simulink model "Sandbox"  (R2026b)
settings: Solver=VariableStepAuto  StopTime=20
model workspace (MAT data in the model file):
  MW_MaxNumBodies = 100
  MW_MaxNumCollisions = 5
  MW_MaxNumVertices = 10000
undefined symbols (not defined in the file): K_Lookup, t_s, Tau_Lookup
libraries: simulink x1, embmathops x1
settings Model: Creator=Janelyn Anderson  LastModifiedBy=Janelyn Anderson
settings SimscapeCC: SimscapeLogType=all  SimscapeNominalValues="[{\"value\":\"1\",\"unit\":\"A\"},{\"value\":\"1\",\"unit\":\"bar\"},{\"value\":\"1\",\"unit\":\"cm^2\"},{\"value\":\"1\",\"unit\":\"cm^3/s\"},{\"value\":\"1\",\"unit\":\"kJ/kg\"},{\"value\":\"1\",\"unit\":\"kW\"},{\"value\":\"1\",\"unit\":\"l\"},{\"value\":\"1\",\"unit\":\"N\"},{\"value\":\"1\",\"unit\":\"N*m\"},{\"value\":\"1\",\"unit\":\"V\"},{\"value\":\"0.001\",\"unit\":\"Wb\"}]"  SimscapeUseEnergyAccounting=off

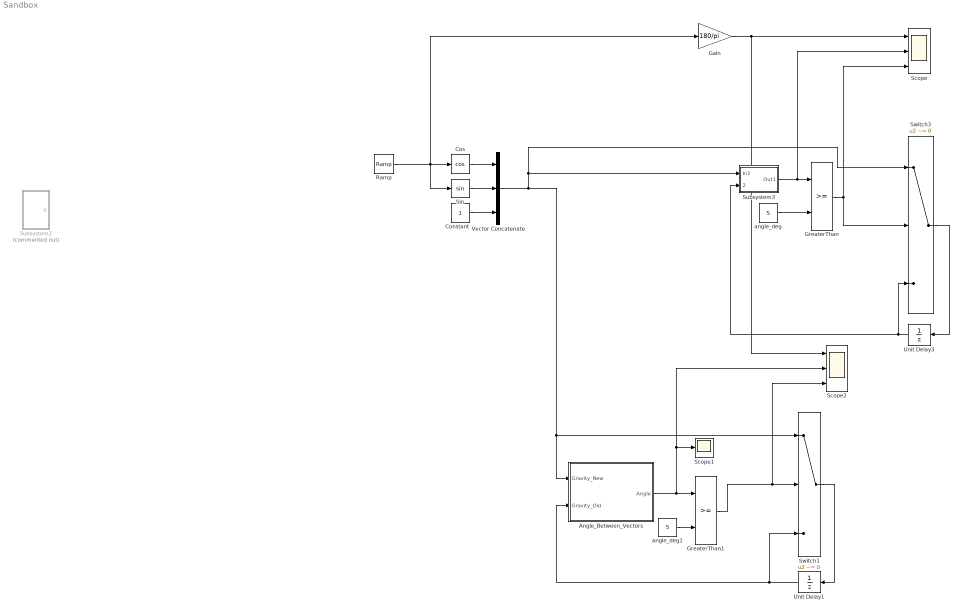
== system Sandbox ==
  Angle_Between_Vectors : Subsystem
  Constant : Constant
  Cos : Trigonometry  Operator=cos
  Gain : Gain  Gain=180/pi
  GreaterThan : RelationalOperator  OutDataTypeStr=boolean  RndMeth=Simplest  InputSameDT=off
  GreaterThan1 : RelationalOperator  OutDataTypeStr=boolean  RndMeth=Simplest  InputSameDT=off
  Ramp : simulink/Sources/Ramp  slope=(10/360)*(2*pi)/20  start=0  InitialOutput=0
  Scope : Scope  NumInputPorts=3
      settings: ActiveDisplayYMinimum=-1.2499999999999998  ActiveDisplayYMaximum=11.25
  Scope1 : Scope
      settings: ActiveDisplayYMinimum=44.999776956803615  ActiveDisplayYMaximum=45.002007388767574
  Scope2 : Scope  NumInputPorts=3
      settings: ActiveDisplayYMinimum=-1.2499999999999998  ActiveDisplayYMaximum=11.25  DataLoggingVariableName=ScopeData2
  Sin : Trigonometry
  Subsystem2 : Subsystem  Commented=on
  Subsystem3 : Subsystem
  Switch1 : Switch  Criteria=u2 ~= 0  SaturateOnIntegerOverflow=off  InputSameDT=off
  Switch3 : Switch  Criteria=u2 ~= 0  SaturateOnIntegerOverflow=off  InputSameDT=off
  Unit Delay1 : UnitDelay  InitialCondition=[1 0 1]  SampleTime=-1
  Unit Delay3 : UnitDelay  InitialCondition=[1 0 1]  SampleTime=-1
  Vector Concatenate : Concatenate  NumInputs=3
  angle_deg : Constant  Value=5
  angle_deg1 : Constant  Value=5
  wires:
  GreaterThan/1 -> Scope/3, Switch3/2
  Switch3/1 -> Unit Delay3/1
  angle_deg/1 -> GreaterThan/2
  Unit Delay3/1 -> Switch3/3, Subsystem3/2(Gravity)
  Cos/1 -> Vector Concatenate/1
  Sin/1 -> Vector Concatenate/2
  Constant/1 -> Vector Concatenate/3
  Ramp/1 -> Sin/1, Gain/1, Cos/1
  Gain/1 -> Scope2/1, Scope/1
  Unit Delay1/1 -> Switch1/3, Angle_Between_Vectors/2(Gravity_Old)
  Switch1/1 -> Unit Delay1/1
  Vector Concatenate/1 -> Angle_Between_Vectors/1(Gravity_New), Switch1/1, Switch3/1, Subsystem3/1(In1)
  Angle_Between_Vectors/1(Angle) -> Scope2/2, Scope1/1, GreaterThan1/1
  angle_deg1/1 -> GreaterThan1/2
  GreaterThan1/1 -> Scope2/3, Switch1/2
  Subsystem3/1(Out1) -> Scope/2, GreaterThan/1

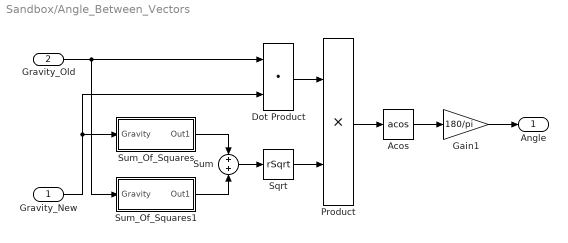
== system Sandbox/Angle_Between_Vectors ==
  Gravity_New : Inport
  Gravity_Old : Inport  Port=2
  Acos : Trigonometry  Operator=acos  OutputSignalType=real
  Dot Product : DotProduct  OutDataTypeStr=Inherit: Inherit via internal rule
  Gain1 : Gain  Gain=180/pi
  Product : Product
  Sqrt : Sqrt  Operator=rSqrt
  Sum : Sum  Inputs=+|+
  Sum_Of_Squares : Subsystem
  Sum_Of_Squares1 : Subsystem
  Angle : Outport
  wires:
  Acos/1 -> Gain1/1
  Sqrt/1 -> Product/2
  Product/1 -> Acos/1
  Dot Product/1 -> Product/1
  Sum_Of_Squares/1(Out1) -> Sum/1
  Gravity_Old/1 -> Dot Product/1, Sum_Of_Squares1/1(Gravity)
  Gravity_New/1 -> Sum_Of_Squares/1(Gravity), Dot Product/2
  Sum/1 -> Sqrt/1
  Sum_Of_Squares1/1(Out1) -> Sum/2
  Gain1/1 -> Angle/1

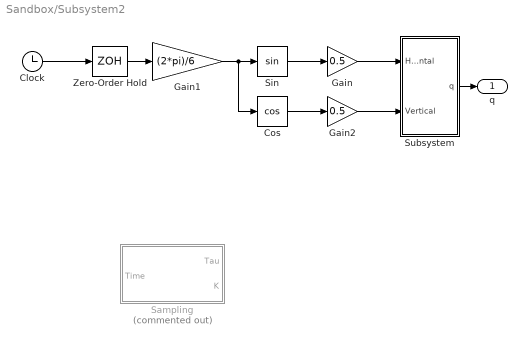
== system Sandbox/Subsystem2 ==
  Clock : Clock
  Cos : Trigonometry  Operator=cos
  Gain : Gain  Gain=0.5
  Gain1 : Gain  Gain=(2*pi)/6
  Gain2 : Gain  Gain=0.5
  Sampling : Subsystem  Commented=on
  Sin : Trigonometry
  Subsystem : Subsystem
  Zero-Order Hold : ZeroOrderHold  SampleTime=t_s
  q : Outport
  wires:
  Cos/1 -> Gain2/1
  Clock/1 -> Zero-Order Hold/1
  Sin/1 -> Gain/1
  Subsystem/1(q) -> q/1
  Zero-Order Hold/1 -> Gain1/1
  Gain1/1 -> Cos/1, Sin/1
  Gain/1 -> Subsystem/1(Horizontal)
  Gain2/1 -> Subsystem/2(Vertical)

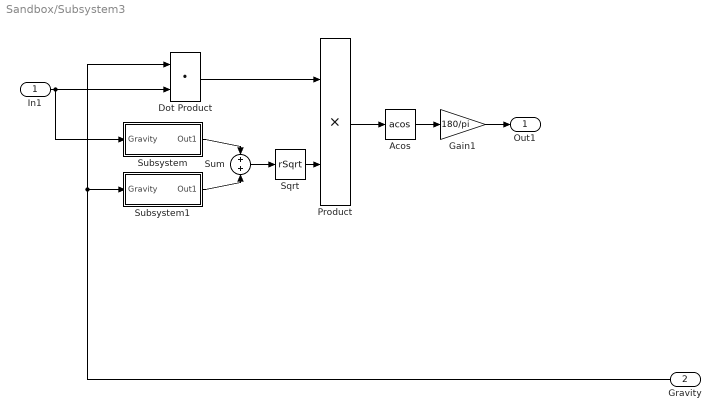
== system Sandbox/Subsystem3 ==
  In1 : Inport
  Gravity : Inport  Port=2
  Acos : Trigonometry  Operator=acos  OutputSignalType=real
  Dot Product : DotProduct  OutDataTypeStr=Inherit: Inherit via internal rule
  Gain1 : Gain  Gain=180/pi
  Product : Product
  Sqrt : Sqrt  Operator=rSqrt
  Subsystem : Subsystem
  Subsystem1 : Subsystem
  Sum : Sum  Inputs=+|+
  Out1 : Outport
  wires:
  Dot Product/1 -> Product/1
  Gravity/1 -> Dot Product/1, Subsystem1/1(Gravity)
  Sum/1 -> Sqrt/1
  Subsystem1/1(Out1) -> Sum/2
  Product/1 -> Acos/1
  Sqrt/1 -> Product/2
  Subsystem/1(Out1) -> Sum/1
  Acos/1 -> Gain1/1
  Gain1/1 -> Out1/1
  In1/1 -> Subsystem/1(Gravity), Dot Product/2

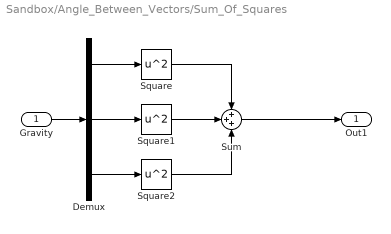
== system Sandbox/Angle_Between_Vectors/Sum_Of_Squares ==
  Gravity : Inport
  Demux : Demux  Outputs=3
  Square : Math  Operator=square
  Square1 : Math  Operator=square
  Square2 : Math  Operator=square
  Sum : Sum  Inputs=+++
  Out1 : Outport
  wires:
  Gravity/1 -> Demux/1
  Demux/3 -> Square2/1
  Demux/2 -> Square1/1
  Demux/1 -> Square/1
  Square1/1 -> Sum/2
  Square/1 -> Sum/1
  Square2/1 -> Sum/3
  Sum/1 -> Out1/1

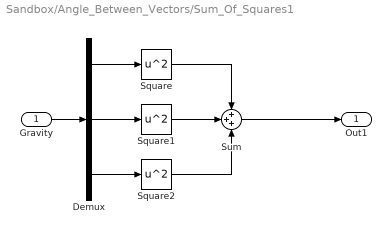
== system Sandbox/Angle_Between_Vectors/Sum_Of_Squares1 ==
  Gravity : Inport
  Demux : Demux  Outputs=3
  Square : Math  Operator=square
  Square1 : Math  Operator=square
  Square2 : Math  Operator=square
  Sum : Sum  Inputs=+++
  Out1 : Outport
  wires:
  Gravity/1 -> Demux/1
  Demux/3 -> Square2/1
  Demux/2 -> Square1/1
  Demux/1 -> Square/1
  Square1/1 -> Sum/2
  Square/1 -> Sum/1
  Square2/1 -> Sum/3
  Sum/1 -> Out1/1

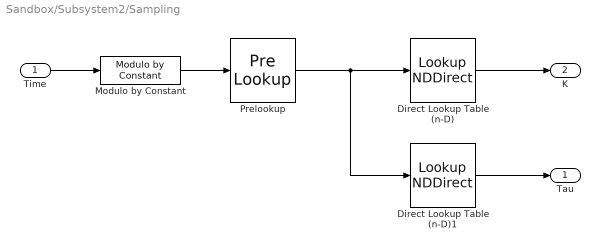
== system Sandbox/Subsystem2/Sampling ==
  Time : Inport
  Direct Lookup Table (n-D) : LookupNDDirect  NumberOfTableDimensions=3  InputsSelectThisObjectFromTable=2-D Matrix  Table=K_Lookup
  Direct Lookup Table (n-D)1 : LookupNDDirect  InputsSelectThisObjectFromTable=Vector  Table=Tau_Lookup
  Modulo by Constant : embmathops/Modulo by Constant  Denominator=3  SimulateUsing=Code generation
      settings: LibrarySourceBlock=embeddedMathLib/Modulo by Constant
  Prelookup : PreLookup  BreakpointsData=T_Breakpoints  OutputSelection=Index only
  Tau : Outport
  K : Outport  Port=2
  wires:
  Modulo by Constant/1 -> Prelookup/1
  Prelookup/1 -> Direct Lookup Table (n-D)1/1, Direct Lookup Table (n-D)/1
  Direct Lookup Table (n-D)/1 -> K/1
  Direct Lookup Table (n-D)1/1 -> Tau/1
  Time/1 -> Modulo by Constant/1

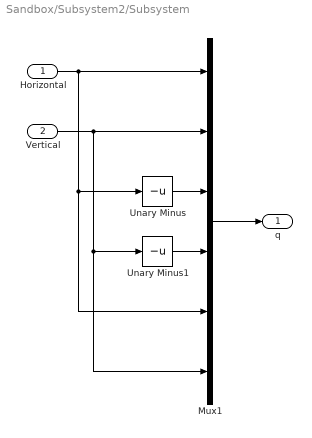
== system Sandbox/Subsystem2/Subsystem ==
  Horizontal : Inport
  Vertical : Inport  Port=2
  Mux1 : Mux  Inputs=6
  Unary Minus : UnaryMinus
  Unary Minus1 : UnaryMinus
  q : Outport
  wires:
  Unary Minus1/1 -> Mux1/4
  Horizontal/1 -> Mux1/5, Unary Minus/1, Mux1/1
  Vertical/1 -> Mux1/2, Unary Minus1/1, Mux1/6
  Mux1/1 -> q/1
  Unary Minus/1 -> Mux1/3

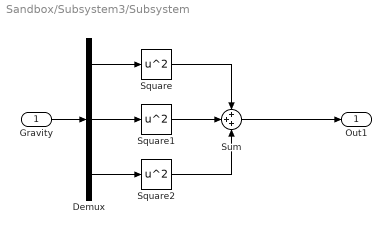
== system Sandbox/Subsystem3/Subsystem ==
  Gravity : Inport
  Demux : Demux  Outputs=3
  Square : Math  Operator=square
  Square1 : Math  Operator=square
  Square2 : Math  Operator=square
  Sum : Sum  Inputs=+++
  Out1 : Outport
  wires:
  Gravity/1 -> Demux/1
  Demux/3 -> Square2/1
  Demux/2 -> Square1/1
  Demux/1 -> Square/1
  Square1/1 -> Sum/2
  Square/1 -> Sum/1
  Square2/1 -> Sum/3
  Sum/1 -> Out1/1

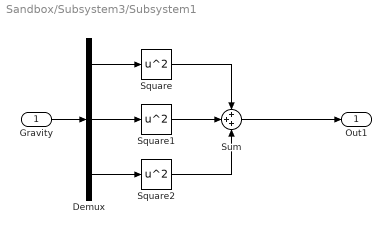
== system Sandbox/Subsystem3/Subsystem1 ==
  Gravity : Inport
  Demux : Demux  Outputs=3
  Square : Math  Operator=square
  Square1 : Math  Operator=square
  Square2 : Math  Operator=square
  Sum : Sum  Inputs=+++
  Out1 : Outport
  wires:
  Gravity/1 -> Demux/1
  Demux/3 -> Square2/1
  Demux/2 -> Square1/1
  Demux/1 -> Square/1
  Square1/1 -> Sum/2
  Square/1 -> Sum/1
  Square2/1 -> Sum/3
  Sum/1 -> Out1/1
